simulink model "Stampfly_Tx"  (R2026b)
settings: Solver=FixedStepDiscrete  StopTime=inf  FixedStep=Official.Step
PostLoadFcn:
  | run(fullfile(fileparts(get_param('Stampfly_Tx','FileName')),'config','startup.m'));
InitFcn:
  | init_imu_flight;
undefined symbols (not defined in the file or in its folder): Official
libraries: slpidlib x7, simulink x4, mspfiltlib x1
(part 3 of 5)

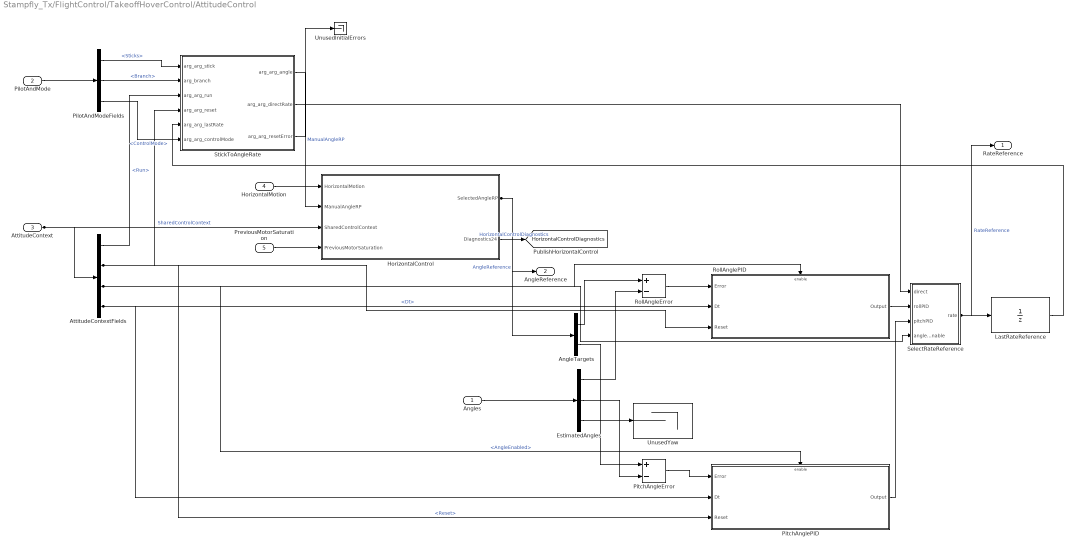
== system Stampfly_Tx/FlightControl/TakeoffHoverControl/AttitudeControl ==
  Angles : Inport
  PilotAndMode : Inport  Port=2
  AttitudeContext : Inport  Port=3
  HorizontalMotion : Inport  Description=HorizontalMotion：水平推定・制御のデータと実行条件を選択・結合します。2軸の順序は局所X（基準機首）、Y（右）です。  Port=4  OutDataTypeStr=Bus: HorizontalMotionBus
  PreviousMotorSaturation : Inport  Description=PreviousMotorSaturation：水平推定・制御のデータと実行条件を選択・結合します。2軸の順序は局所X（基準機首）、Y（右）です。  Port=5  OutDataTypeStr=boolean
  AngleTargets : Demux  Description=AngleTargets：ベクトルを元の成分順に分解します。個別の誤差や符号処理が必要な箇所で使います。  Outputs=2
  AttitudeContextFields : BusSelector  Description=AttitudeContextFields：バスから ControlContext.Run,ControlContext.Reset,ControlContext.AngleEnabled,Dt を選びます。元のベクトルの成分順序は変更しません。  OutputSignals=ControlContext.Run,ControlContext.Reset,ControlContext.AngleEnabled,Dt
  EstimatedAngles : Demux  Description=EstimatedAngles：ベクトルを元の成分順に分解します。個別の誤差や符号処理が必要な箇所で使います。  Outputs=3
  HorizontalControl : Subsystem  Description=HorizontalControl：水平推定・制御のデータと実行条件を選択・結合します。2軸の順序は局所X（基準機首）、Y（右）です。
      mask help: 水平制御：移動・減速・停止位置保持の速度目標、速度PI、姿勢目標への変換を行います。既存の姿勢・角速度PIDの前段です。
      mask Display: disp('HorizontalControl');port_label('input',1,'HorizontalMotion');port_label('input',2,'ManualAngleRP');port_label('input',3,'SharedControlContext');port_label('input',4,'PreviousMotorSaturation');port_label('output',1,'SelectedAngleRP');port_label('output',2,'Diagnostics24');
  LastRateReference : UnitDelay  Description=LastRateReference：前周期の値を保持して出力します。更新順序と状態保持に必要な 1 周期遅延です。初期値 zeros(3,1,'single')、周期 Official.Step 秒。  InitialCondition=zeros(3,1,'single')  SampleTime=Official.Step
  PilotAndModeFields : BusSelector  Description=PilotAndModeFields：バスから PilotInput.Sticks,SharedControlContext.FlightContext.Branch,SharedControlContext.ControlMode を選びます。元のベクトルの成分順序は変更しません。  OutputSignals=PilotInput.Sticks,SharedControlContext.FlightContext.Branch,SharedControlContext.ControlMode
  PitchAngleError : Sum  Description=PitchAngleError：入力を +- の符号で加減算します。ベクトルでは各成分に同じ演算を適用します。  Inputs=+-
  PitchAnglePID : Subsystem  Description=Pitch 角度 PID：角度誤差 [rad]→Pitch 角速度目標 [rad/s]。Stabilize 時の Enabled 境界と低推力 Reset を保ちます。
      mask help: Pitch 角度 PID：角度誤差 [rad]→Pitch 角速度目標 [rad/s]。Stabilize 時の Enabled 境界と低推力 Reset を保ちます。
      mask Display: disp('PitchAnglePID');port_label('input',1,'Error');port_label('input',2,'Dt');port_label('input',3,'Reset');port_label('output',1,'Output');
  RollAngleError : Sum  Description=RollAngleError：入力を +- の符号で加減算します。ベクトルでは各成分に同じ演算を適用します。  Inputs=+-
  RollAnglePID : Subsystem  Description=Roll 角度 PID：角度誤差 [rad]→Roll 角速度目標 [rad/s]。Stabilize 時の Enabled 境界と低推力 Reset を保ちます。
      mask help: Roll 角度 PID：角度誤差 [rad]→Roll 角速度目標 [rad/s]。Stabilize 時の Enabled 境界と低推力 Reset を保ちます。
      mask Display: disp('RollAnglePID');port_label('input',1,'Error');port_label('input',2,'Dt');port_label('input',3,'Reset');port_label('output',1,'Output');
  SelectRateReference : MATLAB Function  Description=角速度 PID の目標 [Roll, Pitch, Yaw] を選びます。Stabilize で角度制御が有効なときだけ Roll/Pitch を角度 PID の出力へ置換し、Yaw と Sport の直接角速度目標はそのまま使います。  TreatAsAtomicUnit=on
  StickToAngleRate : MATLAB Function  Description=操縦スティックから角度・角速度目標を作ります。Stabilize は Roll/Pitch ±30°、Sport は非線形な角速度指令、Yaw は角速度指令です。低推力リセット時に中立値を記憶します。  TreatAsAtomicUnit=on
  UnusedInitialErrors : Terminator
      settings: Description=操縦指令の既存関数が返す初期誤差を終端します。DedicatedPID の Reset により内部誤差を管理します。
  UnusedYaw : Terminator
      settings: Description=UnusedYaw：使用しない観測出力をここで終端します。接続された制御信号を変更しません。
  RateReference : Outport
  AngleReference : Outport  Port=2
  tag scope: HorizontalControlDiagnostics=global
  wires:
  Angles/1 -> EstimatedAngles/1
  AttitudeContextFields/2 -> PitchAnglePID/3(Reset), StickToAngleRate/4(arg_arg_reset), RollAnglePID/3(Reset)  "<Reset>"
  AttitudeContext/1 -> AttitudeContextFields/1, HorizontalControl/3(SharedControlContext)  "SharedControlContext"
  AttitudeContextFields/4 -> PitchAnglePID/2(Dt), RollAnglePID/2(Dt)  "<Dt>"
  PilotAndMode/1 -> PilotAndModeFields/1
  PilotAndModeFields/3 -> StickToAngleRate/6(arg_arg_controlMode)  "<ControlMode>"
  PilotAndModeFields/1 -> StickToAngleRate/1(arg_arg_stick)  "<Sticks>"
  PilotAndModeFields/2 -> StickToAngleRate/2(arg_branch)  "<Branch>"
  AttitudeContextFields/3 -> PitchAnglePID/Enable, SelectRateReference/4(angleEnable), RollAnglePID/Enable  "<AngleEnabled>"
  AttitudeContextFields/1 -> StickToAngleRate/3(arg_arg_run)  "<Run>"
  StickToAngleRate/1(arg_arg_angle) -> HorizontalControl/2(ManualAngleRP)  "ManualAngleRP"
  StickToAngleRate/2(arg_arg_directRate) -> SelectRateReference/1(direct)
  StickToAngleRate/3(arg_arg_resetError) -> UnusedInitialErrors/1
  EstimatedAngles/2 -> PitchAngleError/2
  HorizontalMotion/1 -> HorizontalControl/1(HorizontalMotion)
  RollAnglePID/1(Output) -> SelectRateReference/2(rollPID)
  PreviousMotorSaturation/1 -> HorizontalControl/4(PreviousMotorSaturation)
  HorizontalControl/1(SelectedAngleRP) -> AngleReference/1, AngleTargets/1  "AngleReference"
  HorizontalControl/2(Diagnostics24) -> [HorizontalControlDiagnostics]  "HorizontalControlDiagnostics"
  AngleTargets/1 -> RollAngleError/1
  AngleTargets/2 -> PitchAngleError/1
  SelectRateReference/1(rate) -> LastRateReference/1, RateReference/1  "RateReference"
  EstimatedAngles/1 -> RollAngleError/2
  EstimatedAngles/3 -> UnusedYaw/1
  RollAngleError/1 -> RollAnglePID/1(Error)
  PitchAngleError/1 -> PitchAnglePID/1(Error)
  PitchAnglePID/1(Output) -> SelectRateReference/3(pitchPID)
  LastRateReference/1 -> StickToAngleRate/5(arg_arg_lastRate)

== system Stampfly_Tx/FlightControl/TakeoffHoverControl/BodyRateControl ==
  RateReference : Inport
  MeasuredRates : Inport  Port=2
  RateContext : Inport  Port=3
  EstimatedRates : Demux  Description=EstimatedRates：ベクトルを元の成分順に分解します。個別の誤差や符号処理が必要な箇所で使います。  Outputs=3
  PitchRateError : Sum  Description=PitchRateError：入力を +- の符号で加減算します。ベクトルでは各成分に同じ演算を適用します。  Inputs=+-
  PitchRatePID : Subsystem  Description=Pitch 角速度 PID：角速度誤差 [rad/s]→Pitch のモーター補正。積分状態は Enable と Reset で管理し、実測 dt を入力します。
      mask help: Pitch 角速度 PID：角速度誤差 [rad/s]→Pitch のモーター補正。積分状態は Enable と Reset で管理し、実測 dt を入力します。
      mask Display: disp('PitchRatePID');port_label('input',1,'Error');port_label('input',2,'Dt');port_label('input',3,'Reset');port_label('output',1,'Output');
  RateContextFields : BusSelector  Description=制御の実行・リセット条件と実測 dt を選びます。DedicatedPID 内部で前回誤差を保持するため、未使用の PreviousError は取り出しません。  OutputSignals=ControlContext.Run,ControlContext.Reset,Dt
  RollRateError : Sum  Description=RollRateError：入力を +- の符号で加減算します。ベクトルでは各成分に同じ演算を適用します。  Inputs=+-
  RollRatePID : Subsystem  Description=Roll 角速度 PID：角速度誤差 [rad/s]→Roll のモーター補正。積分状態は Enable と Reset で管理し、実測 dt を入力します。
      mask help: Roll 角速度 PID：角速度誤差 [rad/s]→Roll のモーター補正。積分状態は Enable と Reset で管理し、実測 dt を入力します。
      mask Display: disp('RollRatePID');port_label('input',1,'Error');port_label('input',2,'Dt');port_label('input',3,'Reset');port_label('output',1,'Output');
  TargetRates : Demux  Description=TargetRates：ベクトルを元の成分順に分解します。個別の誤差や符号処理が必要な箇所で使います。  Outputs=3
  YawRateError : Sum  Description=YawRateError：入力を +- の符号で加減算します。ベクトルでは各成分に同じ演算を適用します。  Inputs=+-
  YawRatePID : Subsystem  Description=Yaw 角速度 PID：角速度誤差 [rad/s]→Yaw のモーター補正。Yaw の絶対角度制御は行わず、スティックの角速度目標を使います。
      mask help: Yaw 角速度 PID：角速度誤差 [rad/s]→Yaw のモーター補正。Yaw の絶対角度制御は行わず、スティックの角速度目標を使います。
      mask Display: disp('YawRatePID');port_label('input',1,'Error');port_label('input',2,'Dt');port_label('input',3,'Reset');port_label('output',1,'Output');
  RollTorque : Outport
  PitchTorque : Outport  Port=2
  YawTorque : Outport  Port=3
  wires:
  EstimatedRates/2 -> PitchRateError/2
  MeasuredRates/1 -> EstimatedRates/1
  RateReference/1 -> TargetRates/1
  TargetRates/3 -> YawRateError/1
  TargetRates/1 -> RollRateError/1
  TargetRates/2 -> PitchRateError/1
  EstimatedRates/3 -> YawRateError/2
  EstimatedRates/1 -> RollRateError/2
  RateContext/1 -> RateContextFields/1
  RollRateError/1 -> RollRatePID/1(Error)
  PitchRateError/1 -> PitchRatePID/1(Error)
  YawRateError/1 -> YawRatePID/1(Error)
  RateContextFields/1 -> YawRatePID/Enable, RollRatePID/Enable, PitchRatePID/Enable  "<Run>"
  RateContextFields/2 -> PitchRatePID/3(Reset), RollRatePID/3(Reset), YawRatePID/3(Reset)  "<Reset>"
  RateContextFields/3 -> YawRatePID/2(Dt), RollRatePID/2(Dt), PitchRatePID/2(Dt)  "<Dt>"
  RollRatePID/1(Output) -> RollTorque/1  "RollTorque"
  PitchRatePID/1(Output) -> PitchTorque/1  "PitchTorque"
  YawRatePID/1(Output) -> YawTorque/1  "YawTorque"

== system Stampfly_Tx/FlightControl/TakeoffHoverControl/FlightCommand ==
  PilotInput : Inport
  Height : Inport  Port=2
  FlightContext : Inport  Port=3
  TimingAndThrust : Inport  Port=4
  CommandStatusBus : BusCreator  Description=CommandStatusBus：異なる単位・型を持つ関連信号を名前付きバスにまとめます。入力線の信号名が項目名です。  Inputs=2
  ControlGating : Subsystem  Description=共通推力と飛行分岐から、全体・高度・角度・鉛直速度 PID の実行条件とリセットを決めます。制御の積分状態を校正・待機中に進めないための条件です。
      mask help: 共通推力と飛行分岐から、全体・高度・角度・鉛直速度 PID の実行条件とリセットを決めます。制御の積分状態を校正・待機中に進めないための条件です。
      mask Display: disp('ControlGating');port_label('input',1,'CommandMode');port_label('input',2,'ModeContext');port_label('input',3,'ThrustState');port_label('output',1,'ThrustRequest');port_label('output',2,'ControlContext');
  FinalizeFlightMode : Stateflow chart  Description=離着陸カウンターと制御状態から、周期末のモード・接続状態などを確定します。次周期に渡すモードと最上位の分岐を区別します。  TreatAsAtomicUnit=on
      mask help: 離着陸カウンターと制御状態から、周期末のモード・接続状態などを確定します。次周期に渡すモードと最上位の分岐を区別します。
  FlightCommandBus : BusCreator  Description=FlightCommandBus：異なる単位・型を持つ関連信号を名前付きバスにまとめます。入力線の信号名が項目名です。  Inputs=7
  FlightContextFields : BusSelector  Description=FlightContextFields：バスから Branch,PreMode を選びます。元のベクトルの成分順序は変更しません。  OutputSignals=Branch,PreMode
  ModeContextBus : BusCreator  Description=ModeContextBus：異なる単位・型を持つ関連信号を名前付きバスにまとめます。入力線の信号名が項目名です。  Inputs=3
  PilotInputFields : BusSelector  Description=PilotInputFields：バスから Sticks,BatteryVoltage,RangeFlag,OverG を選びます。元のベクトルの成分順序は変更しません。  OutputSignals=Sticks,BatteryVoltage,RangeFlag,OverG
  SharedControlContextBus : BusCreator  Description=SharedControlContextBus：異なる単位・型を持つ関連信号を名前付きバスにまとめます。入力線の信号名が項目名です。  Inputs=8
  TakeoffLandingCommand : Stateflow chart  Description=離陸・着陸、0.5 m の初期高度目標、0.05～1.8 m の高さ設定、基準推力と電圧トリムを状態として管理する Stateflow です。  TreatAsAtomicUnit=on
      mask help: 離陸・着陸、0.5 m の初期高度目標、0.05～1.8 m の高さ設定、基準推力と電圧トリムを状態として管理する Stateflow です。
  TimingAndThrustFields : BusSelector  Description=TimingAndThrustFields：バスから Dt,ThrustState を選びます。元のベクトルの成分順序は変更しません。  OutputSignals=Dt,ThrustState
  Zero : Constant  Description=Zero：固定値 single(0) を出力します。意味と単位は親の機能説明と信号名を参照します。  Value=single(0)
  FlightCommand : Outport
  SharedControlContext : Outport  Port=2
  CommandStatus : Outport  Port=3
  wires:
  ModeContextBus/1 -> ControlGating/2(ModeContext)  "ModeContext"
  Height/1 -> FinalizeFlightMode/3(height), TakeoffLandingCommand/2(height)
  TimingAndThrust/1 -> TimingAndThrustFields/1
  ControlGating/2(ControlContext) -> SharedControlContextBus/1  "ControlContext"
  PilotInput/1 -> SharedControlContextBus/3, PilotInputFields/1  "PilotInput"
  TakeoffLandingCommand/7(controlMode) -> SharedControlContextBus/8, FlightCommandBus/7  "ControlMode"
  FlightContext/1 -> ModeContextBus/1, SharedControlContextBus/2, FlightContextFields/1  "FlightContext"
  TakeoffLandingCommand/4(raw) -> FlightCommandBus/4  "RawThrust"
  FlightContextFields/1 -> TakeoffLandingCommand/5(mode), FinalizeFlightMode/1(branch)  "<Branch>"
  PilotInputFields/1 -> TakeoffLandingCommand/1(stick)  "<Sticks>"
  TakeoffLandingCommand/5(auto) -> FlightCommandBus/5, CommandStatusBus/1  "AltitudeEnabled"
  FlightContextFields/2 -> FinalizeFlightMode/2(preMode)  "<PreMode>"
  PilotInputFields/2 -> TakeoffLandingCommand/3(voltage)  "<BatteryVoltage>"
  PilotInputFields/3 -> TakeoffLandingCommand/4(rangeFlag)  "<RangeFlag>"
  PilotInputFields/4 -> FinalizeFlightMode/4(overG)  "<OverG>"
  TimingAndThrustFields/1 -> SharedControlContextBus/5, ModeContextBus/3  "<Dt>"
  TimingAndThrustFields/2 -> ControlGating/3(ThrustState)  "<ThrustState>"
  FinalizeFlightMode/1(mode) -> SharedControlContextBus/4, CommandStatusBus/2, ModeContextBus/2  "Mode"
  ControlGating/1(ThrustRequest) -> SharedControlContextBus/7  "ThrustRequest"
  TakeoffLandingCommand/1(alt) -> FlightCommandBus/1  "HeightReference"
  TakeoffLandingCommand/2(base) -> FlightCommandBus/2  "BaseThrust"
  TakeoffLandingCommand/3(counter) -> FlightCommandBus/3  "RampCounter"
  TakeoffLandingCommand/6(manual) -> FlightCommandBus/6  "ManualAltitude"
  FlightCommandBus/1 -> ControlGating/1(CommandMode), FlightCommand/1  "FlightCommand"
  CommandStatusBus/1 -> CommandStatus/1  "CommandStatus"
  Zero/1 -> SharedControlContextBus/6  "PreviousError"
  SharedControlContextBus/1 -> SharedControlContext/1  "SharedControlContext"

== system Stampfly_Tx/FlightControl/TakeoffHoverControl/FlightDiagnostics ==
  FlightCommand : Inport
  ControlReferences : Inport  Port=2
  MotorDiagnostics : Inport  Port=3
  ControlDiagnosticPack : MATLAB Function  Description=制御内部の観測値を 17 要素の single ベクトルにまとめます。ログの項目順は [高度制御状態; 基準推力; 離陸カウンター; 高度目標; 推力; 角度目標2; 角速度目標3; 軸補正3; 配分前モーター値4] です。制御判断は行いません。  TreatAsAtomicUnit=on
  ControlReferencesFields : BusSelector  Description=ControlReferencesFields：バスから VelocityReference,Thrust,Angles,RateReference を選びます。元のベクトルの成分順序は変更しません。  OutputSignals=VelocityReference,Thrust,Angles,RateReference
  FlightCommandFields : BusSelector  Description=FlightCommandFields：バスから HeightReference,BaseThrust,RampCounter を選びます。元のベクトルの成分順序は変更しません。  OutputSignals=HeightReference,BaseThrust,RampCounter
  MotorDiagnosticsFields : BusSelector  Description=MotorDiagnosticsFields：バスから RollTorque,PitchTorque,YawTorque,BeforeLimit を選びます。元のベクトルの成分順序は変更しません。  OutputSignals=RollTorque,PitchTorque,YawTorque,BeforeLimit
  Diagnostics : Outport
  wires:
  MotorDiagnostics/1 -> MotorDiagnosticsFields/1
  FlightCommand/1 -> FlightCommandFields/1
  ControlReferences/1 -> ControlReferencesFields/1
  FlightCommandFields/1 -> ControlDiagnosticPack/1(alt)  "<HeightReference>"
  FlightCommandFields/2 -> ControlDiagnosticPack/2(base)  "<BaseThrust>"
  ControlReferencesFields/1 -> ControlDiagnosticPack/4(zRef)  "<VelocityReference>"
  FlightCommandFields/3 -> ControlDiagnosticPack/3(counter)  "<RampCounter>"
  ControlReferencesFields/2 -> ControlDiagnosticPack/5(thrust)  "<Thrust>"
  ControlReferencesFields/3 -> ControlDiagnosticPack/6(angle)  "<Angles>"
  ControlReferencesFields/4 -> ControlDiagnosticPack/7(rate)  "<RateReference>"
  MotorDiagnosticsFields/1 -> ControlDiagnosticPack/8(rollTorque)  "<RollTorque>"
  MotorDiagnosticsFields/2 -> ControlDiagnosticPack/9(pitchTorque)  "<PitchTorque>"
  MotorDiagnosticsFields/3 -> ControlDiagnosticPack/10(yawTorque)  "<YawTorque>"
  MotorDiagnosticsFields/4 -> ControlDiagnosticPack/11(before)  "<BeforeLimit>"
  ControlDiagnosticPack/1(diag) -> Diagnostics/1  "Diagnostics"

== system Stampfly_Tx/FlightControl/TakeoffHoverControl/JapaneseExplanation ==

== system Stampfly_Tx/FlightControl/TakeoffHoverControl/MotorAllocation ==
  MotorEffort : Inport
  MotorContext : Inport  Port=2
  MotorCommandBus : BusCreator  Description=MotorCommandBus：異なる単位・型を持つ関連信号を名前付きバスにまとめます。入力線の信号名が項目名です。  Inputs=2
  MotorContextFields : BusSelector  Description=MotorContextFields：バスから ControlContext.Run,ControlContext.Reset,PilotInput.OverG,FlightContext.Branch,Dt を選びます。元のベクトルの成分順序は変更しません。  OutputSignals=ControlContext.Run,ControlContext.Reset,PilotInput.OverG,FlightContext.Branch,Dt
  MotorEffortFields : BusSelector  Description=MotorEffortFields：バスから Thrust,RollTorque,PitchTorque,YawTorque を選びます。元のベクトルの成分順序は変更しません。  OutputSignals=Thrust,RollTorque,PitchTorque,YawTorque
  MotorMixerFilter8bit : Subsystem  Description=4 モーターの符号付き配分、平滑化、飽和、8 bit 変換を一連の処理として示します。モーター順 [FR, FL, RR, RL] は出力・ログでも同じです。
      mask help: 4 モーターの符号付き配分、平滑化、飽和、8 bit 変換を一連の処理として示します。モーター順 [FR, FL, RR, RL] は出力・ログでも同じです。
      mask Display: disp('MotorMixerFilter8bit');port_label('input',1,'Thrust');port_label('input',2,'RollTorque');port_label('input',3,'PitchTorque');port_label('input',4,'YawTorque');port_label('input',5,'Run');port_label('input',6,'Reset');port_label('input',7,'OverG');port_label('input',8,'Mode');port_label('input',9,'Dt');port_label('output',1,'Duty4');port_label('output',2,'Counts4');port_label('output',3,'BeforeLimit4');
  MotorCommand : Outport
  BeforeLimit : Outport  Port=2
  wires:
  MotorEffortFields/1 -> MotorMixerFilter8bit/1(Thrust)  "<Thrust>"
  MotorMixerFilter8bit/3(BeforeLimit4) -> BeforeLimit/1  "BeforeLimit"
  MotorEffort/1 -> MotorEffortFields/1
  MotorContextFields/2 -> MotorMixerFilter8bit/6(Reset)  "<Reset>"
  MotorEffortFields/3 -> MotorMixerFilter8bit/3(PitchTorque)  "<PitchTorque>"
  MotorContext/1 -> MotorContextFields/1
  MotorContextFields/1 -> MotorMixerFilter8bit/5(Run)  "<Run>"
  MotorEffortFields/2 -> MotorMixerFilter8bit/2(RollTorque)  "<RollTorque>"
  MotorEffortFields/4 -> MotorMixerFilter8bit/4(YawTorque)  "<YawTorque>"
  MotorContextFields/3 -> MotorMixerFilter8bit/7(OverG)  "<OverG>"
  MotorContextFields/4 -> MotorMixerFilter8bit/8(Mode)  "<Branch>"
  MotorContextFields/5 -> MotorMixerFilter8bit/9(Dt)  "<Dt>"
  MotorMixerFilter8bit/1(Duty4) -> MotorCommandBus/1  "Duty"
  MotorMixerFilter8bit/2(Counts4) -> MotorCommandBus/2  "Counts"
  MotorCommandBus/1 -> MotorCommand/1  "MotorCommand"

== system Stampfly_Tx/SensorCorrection/IMUAxisConversion/JapaneseExplanation ==

== system Stampfly_Tx/SensorCorrection/IMUFiltering/AccelLowpassXYZ ==
  Input : Inport  PortDimensions=3
  Dt : Inport  Port=2
  Reset : Inport  Port=3
  Enable : Inport  Port=4
  Denominator : Sum  Description=Denominator：入力を ++ の符号で加減算します。ベクトルでは各成分に同じ演算を適用します。
  InputTerm : Product  Description=InputTerm：入力の乗算・除算（*/）を行います。フィルターは既存の演算順序を保ちます。  Inputs=*/
  InputTimesDt : Product  Description=InputTimesDt：入力の乗算・除算（**）を行います。フィルターは既存の演算順序を保ちます。  Inputs=**
  PreviousFiltered : UnitDelay  Description=PreviousFiltered：前周期の値を保持して出力します。更新順序と状態保持に必要な 1 周期遅延です。初期値 zeros(3,1,'single')、周期 .0025 秒。  InitialCondition=zeros(3,1,'single')  SampleTime=.0025
  PreviousTerm : Product  Description=PreviousTerm：入力の乗算・除算（*/）を行います。フィルターは既存の演算順序を保ちます。  Inputs=*/
  PreviousTimesT : Product  Description=PreviousTimesT：入力の乗算・除算（**）を行います。フィルターは既存の演算順序を保ちます。  Inputs=**
  ResetPrevious : Switch  Description=ResetPrevious：条件入力で更新値と保持・リセット値を選びます。条件は u2 ~= 0。  Criteria=u2 ~= 0  SaturateOnIntegerOverflow=off  InputSameDT=off
  TimeConstantS : Constant  Description=TimeConstantS：固定値 single(0.0030000000000000001) を出力します。意味と単位は親の機能説明と信号名を参照します。  Value=single(0.0030000000000000001)
  UpdateOrHold : Switch  Description=UpdateOrHold：条件入力で更新値と保持・リセット値を選びます。条件は u2 ~= 0。  Criteria=u2 ~= 0  SaturateOnIntegerOverflow=off  InputSameDT=off
  UpdatedFiltered : Sum  Description=UpdatedFiltered：入力を ++ の符号で加減算します。ベクトルでは各成分に同じ演算を適用します。
  ZeroOnReset : Constant  Description=ZeroOnReset：固定値 zeros(3,1,'single') を出力します。意味と単位は親の機能説明と信号名を参照します。  Value=zeros(3,1,'single')
  Filtered : Outport
  wires:
  Reset/1 -> ResetPrevious/2
  TimeConstantS/1 -> PreviousTimesT/2, Denominator/1
  Input/1 -> InputTimesDt/1
  Enable/1 -> UpdateOrHold/2
  InputTerm/1 -> UpdatedFiltered/2
  Denominator/1 -> PreviousTerm/2, InputTerm/2
  InputTimesDt/1 -> InputTerm/1
  ResetPrevious/1 -> UpdateOrHold/3, PreviousTimesT/1
  Dt/1 -> Denominator/2, InputTimesDt/2
  UpdatedFiltered/1 -> UpdateOrHold/1
  UpdateOrHold/1 -> PreviousFiltered/1, Filtered/1
  ZeroOnReset/1 -> ResetPrevious/1
  PreviousFiltered/1 -> ResetPrevious/3
  PreviousTimesT/1 -> PreviousTerm/1
  PreviousTerm/1 -> UpdatedFiltered/1

== system Stampfly_Tx/SensorCorrection/IMUFiltering/GyroLowpassXYZ ==
  Input : Inport  PortDimensions=3
  Dt : Inport  Port=2
  Reset : Inport  Port=3
  Enable : Inport  Port=4
  Denominator : Sum  Description=Denominator：入力を ++ の符号で加減算します。ベクトルでは各成分に同じ演算を適用します。
  InputTerm : Product  Description=InputTerm：入力の乗算・除算（*/）を行います。フィルターは既存の演算順序を保ちます。  Inputs=*/
  InputTimesDt : Product  Description=InputTimesDt：入力の乗算・除算（**）を行います。フィルターは既存の演算順序を保ちます。  Inputs=**
  PreviousFiltered : UnitDelay  Description=PreviousFiltered：前周期の値を保持して出力します。更新順序と状態保持に必要な 1 周期遅延です。初期値 zeros(3,1,'single')、周期 .0025 秒。  InitialCondition=zeros(3,1,'single')  SampleTime=.0025
  PreviousTerm : Product  Description=PreviousTerm：入力の乗算・除算（*/）を行います。フィルターは既存の演算順序を保ちます。  Inputs=*/
  PreviousTimesT : Product  Description=PreviousTimesT：入力の乗算・除算（**）を行います。フィルターは既存の演算順序を保ちます。  Inputs=**
  ResetPrevious : Switch  Description=ResetPrevious：条件入力で更新値と保持・リセット値を選びます。条件は u2 ~= 0。  Criteria=u2 ~= 0  SaturateOnIntegerOverflow=off  InputSameDT=off
  TimeConstantS : Constant  Description=TimeConstantS：固定値 single(0.0030000000000000001) を出力します。意味と単位は親の機能説明と信号名を参照します。  Value=single(0.0030000000000000001)
  UpdateOrHold : Switch  Description=UpdateOrHold：条件入力で更新値と保持・リセット値を選びます。条件は u2 ~= 0。  Criteria=u2 ~= 0  SaturateOnIntegerOverflow=off  InputSameDT=off
  UpdatedFiltered : Sum  Description=UpdatedFiltered：入力を ++ の符号で加減算します。ベクトルでは各成分に同じ演算を適用します。
  ZeroOnReset : Constant  Description=ZeroOnReset：固定値 zeros(3,1,'single') を出力します。意味と単位は親の機能説明と信号名を参照します。  Value=zeros(3,1,'single')
  Filtered : Outport
  wires:
  Reset/1 -> ResetPrevious/2
  TimeConstantS/1 -> PreviousTimesT/2, Denominator/1
  Input/1 -> InputTimesDt/1
  Enable/1 -> UpdateOrHold/2
  InputTerm/1 -> UpdatedFiltered/2
  Denominator/1 -> PreviousTerm/2, InputTerm/2
  InputTimesDt/1 -> InputTerm/1
  ResetPrevious/1 -> UpdateOrHold/3, PreviousTimesT/1
  Dt/1 -> InputTimesDt/2, Denominator/2
  UpdatedFiltered/1 -> UpdateOrHold/1
  UpdateOrHold/1 -> Filtered/1, PreviousFiltered/1
  ZeroOnReset/1 -> ResetPrevious/1
  PreviousFiltered/1 -> ResetPrevious/3
  PreviousTimesT/1 -> PreviousTerm/1
  PreviousTerm/1 -> UpdatedFiltered/1

== system Stampfly_Tx/SensorCorrection/IMUFiltering/JapaneseExplanation ==

== system Stampfly_Tx/SensorCorrection/IMUFiltering/VerticalDeltaLowpass ==
  Input : Inport
  Dt : Inport  Port=2
  Reset : Inport  Port=3
  Enable : Inport  Port=4
  Denominator : Sum  Description=Denominator：入力を ++ の符号で加減算します。ベクトルでは各成分に同じ演算を適用します。
  InputTerm : Product  Description=InputTerm：入力の乗算・除算（*/）を行います。フィルターは既存の演算順序を保ちます。  Inputs=*/
  InputTimesDt : Product  Description=InputTimesDt：入力の乗算・除算（**）を行います。フィルターは既存の演算順序を保ちます。  Inputs=**
  PreviousFiltered : UnitDelay  Description=PreviousFiltered：前周期の値を保持して出力します。更新順序と状態保持に必要な 1 周期遅延です。初期値 single(0)、周期 .0025 秒。  InitialCondition=single(0)  SampleTime=.0025
  PreviousTerm : Product  Description=PreviousTerm：入力の乗算・除算（*/）を行います。フィルターは既存の演算順序を保ちます。  Inputs=*/
  PreviousTimesT : Product  Description=PreviousTimesT：入力の乗算・除算（**）を行います。フィルターは既存の演算順序を保ちます。  Inputs=**
  ResetPrevious : Switch  Description=ResetPrevious：条件入力で更新値と保持・リセット値を選びます。条件は u2 ~= 0。  Criteria=u2 ~= 0  SaturateOnIntegerOverflow=off  InputSameDT=off
  TimeConstantS : Constant  Description=TimeConstantS：固定値 single(0.10000000000000001) を出力します。意味と単位は親の機能説明と信号名を参照します。  Value=single(0.10000000000000001)
  UpdateOrHold : Switch  Description=UpdateOrHold：条件入力で更新値と保持・リセット値を選びます。条件は u2 ~= 0。  Criteria=u2 ~= 0  SaturateOnIntegerOverflow=off  InputSameDT=off
  UpdatedFiltered : Sum  Description=UpdatedFiltered：入力を ++ の符号で加減算します。ベクトルでは各成分に同じ演算を適用します。
  ZeroOnReset : Constant  Description=ZeroOnReset：固定値 single(0) を出力します。意味と単位は親の機能説明と信号名を参照します。  Value=single(0)
  Filtered : Outport
  wires:
  Reset/1 -> ResetPrevious/2
  TimeConstantS/1 -> PreviousTimesT/2, Denominator/1
  Input/1 -> InputTimesDt/1
  Enable/1 -> UpdateOrHold/2
  InputTerm/1 -> UpdatedFiltered/2
  Denominator/1 -> PreviousTerm/2, InputTerm/2
  InputTimesDt/1 -> InputTerm/1
  ResetPrevious/1 -> UpdateOrHold/3, PreviousTimesT/1
  Dt/1 -> Denominator/2, InputTimesDt/2
  UpdatedFiltered/1 -> UpdateOrHold/1
  UpdateOrHold/1 -> PreviousFiltered/1, Filtered/1
  ZeroOnReset/1 -> ResetPrevious/1
  PreviousFiltered/1 -> ResetPrevious/3
  PreviousTimesT/1 -> PreviousTerm/1
  PreviousTerm/1 -> UpdatedFiltered/1

== system Stampfly_Tx/SensorCorrection/VerticalAcceleration/JapaneseExplanation ==

== system Stampfly_Tx/SensorCorrection/VerticalAcceleration/VerticalLowpass ==
  Input : Inport
  Dt : Inport  Port=2
  Reset : Inport  Port=3
  Enable : Inport  Port=4
  Denominator : Sum  Description=Denominator：入力を ++ の符号で加減算します。ベクトルでは各成分に同じ演算を適用します。
  InputTerm : Product  Description=InputTerm：入力の乗算・除算（*/）を行います。フィルターは既存の演算順序を保ちます。  Inputs=*/
  InputTimesDt : Product  Description=InputTimesDt：入力の乗算・除算（**）を行います。フィルターは既存の演算順序を保ちます。  Inputs=**
  PreviousFiltered : UnitDelay  Description=PreviousFiltered：前周期の値を保持して出力します。更新順序と状態保持に必要な 1 周期遅延です。初期値 single(0)、周期 .0025 秒。  InitialCondition=single(0)  SampleTime=.0025
  PreviousTerm : Product  Description=PreviousTerm：入力の乗算・除算（*/）を行います。フィルターは既存の演算順序を保ちます。  Inputs=*/
  PreviousTimesT : Product  Description=PreviousTimesT：入力の乗算・除算（**）を行います。フィルターは既存の演算順序を保ちます。  Inputs=**
  ResetPrevious : Switch  Description=ResetPrevious：条件入力で更新値と保持・リセット値を選びます。条件は u2 ~= 0。  Criteria=u2 ~= 0  SaturateOnIntegerOverflow=off  InputSameDT=off
  TimeConstantS : Constant  Description=TimeConstantS：固定値 single(0.10000000000000001) を出力します。意味と単位は親の機能説明と信号名を参照します。  Value=single(0.10000000000000001)
  UpdateOrHold : Switch  Description=UpdateOrHold：条件入力で更新値と保持・リセット値を選びます。条件は u2 ~= 0。  Criteria=u2 ~= 0  SaturateOnIntegerOverflow=off  InputSameDT=off
  UpdatedFiltered : Sum  Description=UpdatedFiltered：入力を ++ の符号で加減算します。ベクトルでは各成分に同じ演算を適用します。
  ZeroOnReset : Constant  Description=ZeroOnReset：固定値 single(0) を出力します。意味と単位は親の機能説明と信号名を参照します。  Value=single(0)
  Filtered : Outport
  wires:
  Reset/1 -> ResetPrevious/2
  TimeConstantS/1 -> Denominator/1, PreviousTimesT/2
  Input/1 -> InputTimesDt/1
  Enable/1 -> UpdateOrHold/2
  InputTerm/1 -> UpdatedFiltered/2
  Denominator/1 -> PreviousTerm/2, InputTerm/2
  InputTimesDt/1 -> InputTerm/1
  ResetPrevious/1 -> UpdateOrHold/3, PreviousTimesT/1
  Dt/1 -> InputTimesDt/2, Denominator/2
  UpdatedFiltered/1 -> UpdateOrHold/1
  UpdateOrHold/1 -> PreviousFiltered/1, Filtered/1
  ZeroOnReset/1 -> ResetPrevious/1
  PreviousFiltered/1 -> ResetPrevious/3
  PreviousTimesT/1 -> PreviousTerm/1
  PreviousTerm/1 -> UpdatedFiltered/1

== system Stampfly_Tx/AttitudeAltitudeEstimation/IMUAttitude/FusionState/UpdateWhenReady ==
  Accel : Inport  PortDimensions=[1 3]
  Gyro : Inport  Port=2  PortDimensions=[1 3]
  Reset : ResetPort  DisableCoverage=on  ResetTriggerType=level
  IMU Filter : mspfiltlib/IMU Filter  DispRefFrame=NED  OrientationFormat=quaternion  DecimationFactor=1  InitialProcessNoise=IMUFlight.InitialProcessNoise  AccelerometerNoise=IMUFlight.AccelerometerNoise  GyroscopeNoise=IMUFlight.GyroscopeNoise  GyroscopeDriftNoise=IMUFlight.GyroscopeDriftNoise  LinearAccelerationNoise=IMUFlight.LinearAccelerationNoise  LinearAccelerationDecayFactor=IMUFlight.LinearAccelerationDecayFactor  SimulateUsing=Code generation
  Orientation : Outport  PortDimensions=[1 4]  InitialOutput=single([1 0 0 0])
  AngularVelocity : Outport  Port=2  PortDimensions=[1 3]  InitialOutput=single([0 0 0])
  wires:
  IMU Filter/2 -> AngularVelocity/1
  IMU Filter/1 -> Orientation/1
  Gyro/1 -> IMU Filter/2
  Accel/1 -> IMU Filter/1

== system Stampfly_Tx/FlightControl/TakeoffHoverControl/AltitudeControl/AltitudePID ==
  Error : Inport
  Dt : Inport  Port=2
  Reset : Inport  Port=3
  Enable : EnablePort
  DedicatedPID : slpidlib/PID Controller  Description=飛行比較用の専用PID。Ideal形式、台形積分・微分フィルター、実測Dt、単精度。  Controller=PID  Form=Ideal  TimeDomain=Discrete-time  UseExternalTs=on  SampleTime=.0025  IntegratorMethod=Trapezoidal  FilterMethod=Trapezoidal  ControllerParametersSource=internal  P=single(0.37999999523162842)  I=single(1)/single(10)  UseKiTs=off  D=single(0.5)  UseExternalDerivativeSource=off  N=single(1)/(single(0.125)*single(0.5))  UseFilter=on  TunerSelectOption=Transfer Function Based (PID Tuner App)  InitialConditionSource=external  InitialConditionForIntegrator=0  InitialConditionForFilter=0  DifferentiatorICPrevScaledInput=0  ExternalReset=level  TrackingMode=off  Kt=1  LimitOutput=off  SatLimitsSource=internal  UpperSaturationLimit=inf  LowerSaturationLimit=-inf  LinearizeAsGain=off  AntiWindupMode=none  Kb=1  LimitIntegrator=on  UpperIntegratorSaturationLimit=single(30000)  LowerIntegratorSaturationLimit=single(-30000)  PGainOutDataTypeStr=single  PProdOutDataTypeStr=single  POutMin=[]  POutMax=[]  IGainOutDataTypeStr=single  IProdOutDataTypeStr=single  IOutMin=[]  IOutMax=[]  DGainOutDataTypeStr=single  DProdOutDataTypeStr=single  DOutMin=[]  DOutMax=[]  NGainOutDataTypeStr=single  NProdOutDataTypeStr=single  NOutMin=[]  NOutMax=[]  SumOutDataTypeStr=single  SumOutMin=[]  SumOutMax=[]  SaturationOutDataTypeStr=single  SaturationOutMin=[]  SaturationOutMax=[]  PParamDataTypeStr=single  PParamMin=[]  PParamMax=[]  IParamDataTypeStr=single  IParamMin=[]  IParamMax=[]  DParamDataTypeStr=single  DParamMin=[]  DParamMax=[]  NParamDataTypeStr=single  NParamMin=[]  NParamMax=[]  KbParamDataTypeStr=single  KbParamMin=[]  KbParamMax=[]  KtParamDataTypeStr=single  KtParamMin=[]  KtParamMax=[]  KbOutDataTypeStr=single  KbOutMin=[]  KbOutMax=[]  KtOutDataTypeStr=single  KtOutMin=[]  KtOutMax=[]  IntegratorOutDataTypeStr=single  IntegratorOutMin=[]  IntegratorOutMax=[]  FilterOutDataTypeStr=single  FilterOutMin=[]  FilterOutMax=[]  SumI1OutDataTypeStr=single  SumI1OutMin=[]  SumI1OutMax=[]  SumI2OutDataTypeStr=single  SumI2OutMin=[]  SumI2OutMax=[]  SumI3OutDataTypeStr=single  SumI3OutMin=[]  SumI3OutMax=[]  SumI4OutDataTypeStr=single  SumI4OutMin=[]  SumI4OutMax=[]  SumDOutDataTypeStr=single  SumDOutMin=[]  SumDOutMax=[]  SumAccumDataTypeStr=single  SumI1AccumDataTypeStr=single  SumI2AccumDataTypeStr=single  SumI3AccumDataTypeStr=single  SumI4AccumDataTypeStr=single  SumDAccumDataTypeStr=single  DifferentiatorOutDataTypeStr=single  DifferentiatorOutMin=[]  DifferentiatorOutMax=[]  FilterDiffOutCoefMin=[]  FilterDiffOutCoefMax=[]  ReciprocalOutDataTypeStr=single  ReciprocalOutMin=[]  ReciprocalOutMax=[]  SumDenOutDataTypeStr=single  SumDenOutMin=[]  SumDenOutMax=[]  SumNumOutDataTypeStr=single  SumNumOutMin=[]  SumNumOutMax=[]  SumDenAccumDataTypeStr=single  SumNumAccumDataTypeStr=single  DivideOutDataTypeStr=single  DivideOutMin=[]  DivideOutMax=[]  UdiffTsProdOutDataTypeStr=single  UdiffTsProdOutMin=[]  UdiffTsProdOutMax=[]  NTsProdOutDataTypeStr=single  NTsProdOutMin=[]  NTsProdOutMax=[]  UintegralTsProdOutDataTypeStr=single  UintegralTsProdOutMin=[]  UintegralTsProdOutMax=[]  UngainTsProdOutDataTypeStr=single  UngainTsProdOutMin=[]  UngainTsProdOutMax=[]  ClampingZeroOutDataTypeStr=single  ClampingZeroOutMin=[]  ClampingZeroOutMax=[]  FilterDenConstantOutDataTypeStr=single  FilterDenConstantOutMin=[]  FilterDenConstantOutMax=[]  PCopyOutDataTypeStr=single  PCopyOutMin=[]  PCopyOutMax=[]  NCopyOutDataTypeStr=single  NCopyOutMin=[]  NCopyOutMax=[]  IntegratorContinuousStateAttributes=''  IntegratorStateMustResolveToSignalObject=off  IntegratorRTWStateStorageClass=Auto  FilterContinuousStateAttributes=''  FilterStateMustResolveToSignalObject=off  FilterRTWStateStorageClass=Auto  ParallelPVariant=Passthrough  IdealPVariant=InternalParameters  IVariant=InternalParameters  DVariant=InternalParameters  IntegratorVariant=Discrete  SatVariant=Disabled  AWVariant=Passthrough  PCopyVariant=Disabled  TRVariant=Disabled  FdbkBlocksVariant=Forward  IdealPFdbkVariant=Disabled  SatFdbkVariant=Disabled  DerivativeFilterVariant=TrapezoidalFilter  NVariant=InternalParameters  NCopyVariant=InternalParameters  FilterICVariant=ExternalICs  IntegratorICVariant=ExternalICs  ExternalResetVariant=ExternalReset  TRSumVariant=Passthrough  SumFdbkVariant=Disabled  SumVariant=Sum_PID  TsampFilterVariant=ExternalTs  TsampNgainVariant=Passthrough  TsampIntegralVariant=ExternalTs  ExternalSaturationOutDataTypeStr=Inherit: Same as second input  DerivativeSourceVariant=ErrorSignal  PreIntVariant=InternalPreInt
      settings: LibrarySourceBlock=simulink/Discrete/Discrete PID Controller
  ZeroInitialCondition : Constant  Description=ZeroInitialCondition：固定値 single(0) を出力します。意味と単位は親の機能説明と信号名を参照します。  Value=single(0)
  Output : Outport
  wires:
  DedicatedPID/1 -> Output/1
  Dt/1 -> DedicatedPID/5
  ZeroInitialCondition/1 -> DedicatedPID/3, DedicatedPID/4
  Reset/1 -> DedicatedPID/2
  Error/1 -> DedicatedPID/1

== system Stampfly_Tx/FlightControl/TakeoffHoverControl/AltitudeControl/VerticalSpeedPID ==
  Error : Inport
  Dt : Inport  Port=2
  Reset : Inport  Port=3
  Enable : EnablePort
  DedicatedPID : slpidlib/PID Controller  Description=飛行比較用の専用PID。Ideal形式、台形積分・微分フィルター、実測Dt、単精度。  Controller=PID  Form=Ideal  TimeDomain=Discrete-time  UseExternalTs=on  SampleTime=.0025  IntegratorMethod=Trapezoidal  FilterMethod=Trapezoidal  ControllerParametersSource=internal  P=single(0.079999998211860657)  I=single(1)/single(0.94999998807907104)  UseKiTs=off  D=single(0.079999998211860657)  UseExternalDerivativeSource=off  N=single(1)/(single(0.125)*single(0.079999998211860657))  UseFilter=on  TunerSelectOption=Transfer Function Based (PID Tuner App)  InitialConditionSource=external  InitialConditionForIntegrator=0  InitialConditionForFilter=0  DifferentiatorICPrevScaledInput=0  ExternalReset=level  TrackingMode=off  Kt=1  LimitOutput=off  SatLimitsSource=internal  UpperSaturationLimit=inf  LowerSaturationLimit=-inf  LinearizeAsGain=off  AntiWindupMode=none  Kb=1  LimitIntegrator=on  UpperIntegratorSaturationLimit=single(30000)  LowerIntegratorSaturationLimit=single(-30000)  PGainOutDataTypeStr=single  PProdOutDataTypeStr=single  POutMin=[]  POutMax=[]  IGainOutDataTypeStr=single  IProdOutDataTypeStr=single  IOutMin=[]  IOutMax=[]  DGainOutDataTypeStr=single  DProdOutDataTypeStr=single  DOutMin=[]  DOutMax=[]  NGainOutDataTypeStr=single  NProdOutDataTypeStr=single  NOutMin=[]  NOutMax=[]  SumOutDataTypeStr=single  SumOutMin=[]  SumOutMax=[]  SaturationOutDataTypeStr=single  SaturationOutMin=[]  SaturationOutMax=[]  PParamDataTypeStr=single  PParamMin=[]  PParamMax=[]  IParamDataTypeStr=single  IParamMin=[]  IParamMax=[]  DParamDataTypeStr=single  DParamMin=[]  DParamMax=[]  NParamDataTypeStr=single  NParamMin=[]  NParamMax=[]  KbParamDataTypeStr=single  KbParamMin=[]  KbParamMax=[]  KtParamDataTypeStr=single  KtParamMin=[]  KtParamMax=[]  KbOutDataTypeStr=single  KbOutMin=[]  KbOutMax=[]  KtOutDataTypeStr=single  KtOutMin=[]  KtOutMax=[]  IntegratorOutDataTypeStr=single  IntegratorOutMin=[]  IntegratorOutMax=[]  FilterOutDataTypeStr=single  FilterOutMin=[]  FilterOutMax=[]  SumI1OutDataTypeStr=single  SumI1OutMin=[]  SumI1OutMax=[]  SumI2OutDataTypeStr=single  SumI2OutMin=[]  SumI2OutMax=[]  SumI3OutDataTypeStr=single  SumI3OutMin=[]  SumI3OutMax=[]  SumI4OutDataTypeStr=single  SumI4OutMin=[]  SumI4OutMax=[]  SumDOutDataTypeStr=single  SumDOutMin=[]  SumDOutMax=[]  SumAccumDataTypeStr=single  SumI1AccumDataTypeStr=single  SumI2AccumDataTypeStr=single  SumI3AccumDataTypeStr=single  SumI4AccumDataTypeStr=single  SumDAccumDataTypeStr=single  DifferentiatorOutDataTypeStr=single  DifferentiatorOutMin=[]  DifferentiatorOutMax=[]  FilterDiffOutCoefMin=[]  FilterDiffOutCoefMax=[]  ReciprocalOutDataTypeStr=single  ReciprocalOutMin=[]  ReciprocalOutMax=[]  SumDenOutDataTypeStr=single  SumDenOutMin=[]  SumDenOutMax=[]  SumNumOutDataTypeStr=single  SumNumOutMin=[]  SumNumOutMax=[]  SumDenAccumDataTypeStr=single  SumNumAccumDataTypeStr=single  DivideOutDataTypeStr=single  DivideOutMin=[]  DivideOutMax=[]  UdiffTsProdOutDataTypeStr=single  UdiffTsProdOutMin=[]  UdiffTsProdOutMax=[]  NTsProdOutDataTypeStr=single  NTsProdOutMin=[]  NTsProdOutMax=[]  UintegralTsProdOutDataTypeStr=single  UintegralTsProdOutMin=[]  UintegralTsProdOutMax=[]  UngainTsProdOutDataTypeStr=single  UngainTsProdOutMin=[]  UngainTsProdOutMax=[]  ClampingZeroOutDataTypeStr=single  ClampingZeroOutMin=[]  ClampingZeroOutMax=[]  FilterDenConstantOutDataTypeStr=single  FilterDenConstantOutMin=[]  FilterDenConstantOutMax=[]  PCopyOutDataTypeStr=single  PCopyOutMin=[]  PCopyOutMax=[]  NCopyOutDataTypeStr=single  NCopyOutMin=[]  NCopyOutMax=[]  IntegratorContinuousStateAttributes=''  IntegratorStateMustResolveToSignalObject=off  IntegratorRTWStateStorageClass=Auto  FilterContinuousStateAttributes=''  FilterStateMustResolveToSignalObject=off  FilterRTWStateStorageClass=Auto  ParallelPVariant=Passthrough  IdealPVariant=InternalParameters  IVariant=InternalParameters  DVariant=InternalParameters  IntegratorVariant=Discrete  SatVariant=Disabled  AWVariant=Passthrough  PCopyVariant=Disabled  TRVariant=Disabled  FdbkBlocksVariant=Forward  IdealPFdbkVariant=Disabled  SatFdbkVariant=Disabled  DerivativeFilterVariant=TrapezoidalFilter  NVariant=InternalParameters  NCopyVariant=InternalParameters  FilterICVariant=ExternalICs  IntegratorICVariant=ExternalICs  ExternalResetVariant=ExternalReset  TRSumVariant=Passthrough  SumFdbkVariant=Disabled  SumVariant=Sum_PID  TsampFilterVariant=ExternalTs  TsampNgainVariant=Passthrough  TsampIntegralVariant=ExternalTs  ExternalSaturationOutDataTypeStr=Inherit: Same as second input  DerivativeSourceVariant=ErrorSignal  PreIntVariant=InternalPreInt
      settings: LibrarySourceBlock=simulink/Discrete/Discrete PID Controller
  ZeroInitialCondition : Constant  Description=ZeroInitialCondition：固定値 single(0) を出力します。意味と単位は親の機能説明と信号名を参照します。  Value=single(0)
  Output : Outport
  wires:
  DedicatedPID/1 -> Output/1
  Dt/1 -> DedicatedPID/5
  ZeroInitialCondition/1 -> DedicatedPID/4, DedicatedPID/3
  Reset/1 -> DedicatedPID/2
  Error/1 -> DedicatedPID/1

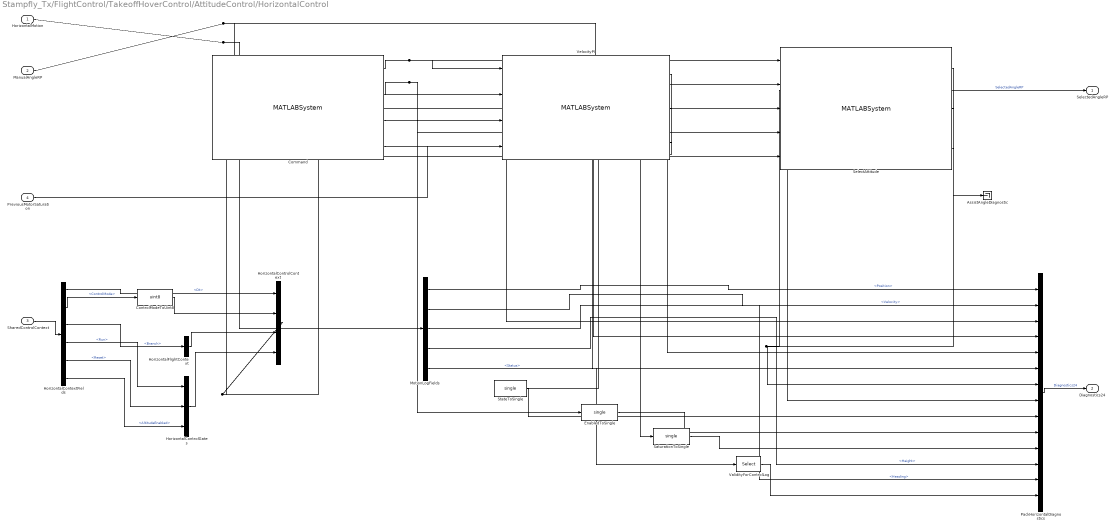
== system Stampfly_Tx/FlightControl/TakeoffHoverControl/AttitudeControl/HorizontalControl ==
  HorizontalMotion : Inport  Description=HorizontalMotion：水平推定・制御のデータと実行条件を選択・結合します。2軸の順序は局所X（基準機首）、Y（右）です。
  ManualAngleRP : Inport  Description=ManualAngleRP：水平推定・制御のデータと実行条件を選択・結合します。2軸の順序は局所X（基準機首）、Y（右）です。  Port=2
  SharedControlContext : Inport  Description=SharedControlContext：水平推定・制御のデータと実行条件を選択・結合します。2軸の順序は局所X（基準機首）、Y（右）です。  Port=3
  PreviousMotorSaturation : Inport  Description=PreviousMotorSaturation：水平推定・制御のデータと実行条件を選択・結合します。2軸の順序は局所X（基準機首）、Y（右）です。  Port=4
  AssistAngleDiagnostic : Terminator
      settings: Description=AssistAngleDiagnostic：水平推定・制御のデータと実行条件を選択・結合します。2軸の順序は局所X（基準機首）、Y（右）です。
  Command : MATLABSystem  Description=|  System=horizontal.Command  Enabled=true  SampleTime=.0025  MaxSpeedMps=.3  CommandAccelerationMps2=.6  PositionGainPerS=.8  EngageHeightM=.20  ReleaseHeightM=.15  HealthyTimeS=.5  RecoveryTimeS=1.0  NeutralEnter=.05  NeutralExit=.08  StopSpeedMps=.08  StopTimeS=.3  ManualAngleLimitRad=pi / 6  SimulateUsing=Code generation
      | %COMMAND 概要：移動・減速・停止位置保持を切り替えて水平速度目標を作ります。
      |     % 既存のスティック中立補正済み角度を、水平補助中だけ速度指令へ解釈します。
      |     % 将来の自動移動は、この出力と同じ局所速度[m/s]を制御器へ渡せます。
      mask Type: horizontal.Command
  ControlModeToUint8 : DataTypeConversion  Description=ControlModeToUint8：水平推定・制御のデータと実行条件を選択・結合します。2軸の順序は局所X（基準機首）、Y（右）です。  OutDataTypeStr=uint8  SaturateOnIntegerOverflow=off  RndMeth=Floor
  EnabledToSingle : DataTypeConversion  Description=EnabledToSingle：水平推定・制御のデータと実行条件を選択・結合します。2軸の順序は局所X（基準機首）、Y（右）です。  OutDataTypeStr=single  SaturateOnIntegerOverflow=off  RndMeth=Floor
  HorizontalContextFields : BusSelector  Description=HorizontalContextFields：水平推定・制御のデータと実行条件を選択・結合します。2軸の順序は局所X（基準機首）、Y（右）です。  OutputSignals=Dt,ControlMode,FlightContext.Branch,ControlContext.Run,ControlContext.Reset,ControlContext.AltitudeEnabled
  HorizontalControlContext : BusCreator  Description=HorizontalControlContext：水平推定・制御のデータと実行条件を選択・結合します。2軸の順序は局所X（基準機首）、Y（右）です。  Inputs=4  OutDataTypeStr=Bus: HorizontalControlContextBus  NonVirtualBus=on
      settings: InheritFromInputs=off
  HorizontalControlGates : BusCreator  Description=HorizontalControlGates：水平推定・制御のデータと実行条件を選択・結合します。2軸の順序は局所X（基準機首）、Y（右）です。  Inputs=3  OutDataTypeStr=Bus: HorizontalControlGatesBus  NonVirtualBus=on
      settings: InheritFromInputs=off
  HorizontalFlightContext : BusCreator  Description=HorizontalFlightContext：水平推定・制御のデータと実行条件を選択・結合します。2軸の順序は局所X（基準機首）、Y（右）です。  Inputs=1  OutDataTypeStr=Bus: HorizontalFlightContextBus  NonVirtualBus=on
      settings: InheritFromInputs=off
  MotionLogFields : BusSelector  Description=MotionLogFields：水平推定・制御のデータと実行条件を選択・結合します。2軸の順序は局所X（基準機首）、Y（右）です。  OutputSignals=Position,Velocity,Heading,Height,Status
  PackHorizontalDiagnostics : Mux  Description=PackHorizontalDiagnostics：水平推定・制御のデータと実行条件を選択・結合します。2軸の順序は局所X（基準機首）、Y（右）です。  Inputs=14
  SaturationToSingle : DataTypeConversion  Description=SaturationToSingle：水平推定・制御のデータと実行条件を選択・結合します。2軸の順序は局所X（基準機首）、Y（右）です。  OutDataTypeStr=single  SaturateOnIntegerOverflow=off  RndMeth=Floor
  SelectAttitude : MATLABSystem  Description=|  System=horizontal.SelectAttitude  SampleTime=.0025  EngageTimeS=.3  ReleaseTimeS=.15  MaxAssistTiltDeg=10  MaxAssistTiltRateDegps=20  SimulateUsing=Code generation
      | %SELECTATTITUDE 概要：水平補助と従来の姿勢目標を滑らかに切り替えます。
      |     % 補助OFFでBlend=0なら元のsingle値をそのまま返し、従来出力を保ちます。
      |             % 1. 有効な水平加速度を、既存の制御座標のRoll/Pitchへ戻します。
      mask Type: horizontal.SelectAttitude
  StateToSingle : DataTypeConversion  Description=StateToSingle：水平推定・制御のデータと実行条件を選択・結合します。2軸の順序は局所X（基準機首）、Y（右）です。  OutDataTypeStr=single  SaturateOnIntegerOverflow=off  RndMeth=Floor
  ValidityForControlLog : Selector  Description=ValidityForControlLog：水平推定・制御のデータと実行条件を選択・結合します。2軸の順序は局所X（基準機首）、Y（右）です。  InputPortWidth=8  IndexOptions=Index vector (dialog)  Indices=[1 4 5 7]  OutputSizes=1
  VelocityPI : MATLABSystem  Description=|  System=horizontal.VelocityPI  SampleTime=.0025  ProportionalGainPerS=1.8  IntegralGainPerS2=.5  MaxAccelerationMps2=.6  IntegralLimitMps2=.25  AccelerationSlewMps3=2.0  SimulateUsing=Code generation
      | %VELOCITYPI 概要：局所水平速度の誤差をPIで水平加速度へ変換します。
      |     % 50 Hzの有効な観測だけ積分し、欠測・解除時は積分をリセットします。
      |     % 速度指令の出所を持たないため、将来の自動移動にも同じ境界を使えます。
      mask Type: horizontal.VelocityPI
  SelectedAngleRP : Outport  Description=SelectedAngleRP：水平推定・制御のデータと実行条件を選択・結合します。2軸の順序は局所X（基準機首）、Y（右）です。
  Diagnostics24 : Outport  Description=Diagnostics24：水平推定・制御のデータと実行条件を選択・結合します。2軸の順序は局所X（基準機首）、Y（右）です。  Port=2
  wires:
  SharedControlContext/1 -> HorizontalContextFields/1
  MotionLogFields/5 -> ValidityForControlLog/1  "<Status>"
  ControlModeToUint8/1 -> HorizontalControlContext/2
  HorizontalContextFields/5 -> HorizontalControlGates/2  "<Reset>"
  Command/1 -> PackHorizontalDiagnostics/3, VelocityPI/1
  HorizontalContextFields/3 -> HorizontalFlightContext/1  "<Branch>"
  PackHorizontalDiagnostics/1 -> Diagnostics24/1  "Diagnostics24"
  HorizontalContextFields/1 -> HorizontalControlContext/1  "<Dt>"
  Command/2 -> EnabledToSingle/1, SelectAttitude/4, VelocityPI/3
  HorizontalContextFields/6 -> HorizontalControlGates/3  "<AltitudeEnabled>"
  HorizontalContextFields/4 -> HorizontalControlGates/1  "<Run>"
  HorizontalControlGates/1 -> HorizontalControlContext/4
  HorizontalContextFields/2 -> ControlModeToUint8/1  "<ControlMode>"
  Command/3 -> StateToSingle/1
  HorizontalFlightContext/1 -> HorizontalControlContext/3
  ManualAngleRP/1 -> SelectAttitude/1, Command/2
  HorizontalMotion/1 -> SelectAttitude/3, MotionLogFields/1, VelocityPI/2, Command/1
  HorizontalControlContext/1 -> SelectAttitude/5, Command/3
  MotionLogFields/2 -> PackHorizontalDiagnostics/2  "<Velocity>"
  Command/4 -> PackHorizontalDiagnostics/4
  MotionLogFields/1 -> PackHorizontalDiagnostics/1  "<Position>"
  EnabledToSingle/1 -> PackHorizontalDiagnostics/10
  PreviousMotorSaturation/1 -> VelocityPI/4
  VelocityPI/1 -> PackHorizontalDiagnostics/5, SelectAttitude/2
  VelocityPI/2 -> PackHorizontalDiagnostics/6
  VelocityPI/3 -> SaturationToSingle/1
  MotionLogFields/3 -> PackHorizontalDiagnostics/13  "<Heading>"
  MotionLogFields/4 -> PackHorizontalDiagnostics/12  "<Height>"
  StateToSingle/1 -> PackHorizontalDiagnostics/9
  SaturationToSingle/1 -> PackHorizontalDiagnostics/11
  SelectAttitude/1 -> SelectedAngleRP/1, PackHorizontalDiagnostics/7  "SelectedAngleRP"
  SelectAttitude/2 -> PackHorizontalDiagnostics/8
  SelectAttitude/3 -> AssistAngleDiagnostic/1
  ValidityForControlLog/1 -> PackHorizontalDiagnostics/14

== system Stampfly_Tx/FlightControl/TakeoffHoverControl/AttitudeControl/PitchAnglePID ==
  Error : Inport
  Dt : Inport  Port=2
  Reset : Inport  Port=3
  Enable : EnablePort
  DedicatedPID : slpidlib/PID Controller  Description=飛行比較用の専用PID。Ideal形式、台形積分・微分フィルター、実測Dt、単精度。  Controller=PID  Form=Ideal  TimeDomain=Discrete-time  UseExternalTs=on  SampleTime=.0025  IntegratorMethod=Trapezoidal  FilterMethod=Trapezoidal  ControllerParametersSource=internal  P=single(5)  I=single(1)/single(4)  UseKiTs=off  D=single(0.039999999105930328)  UseExternalDerivativeSource=off  N=single(1)/(single(0.125)*single(0.039999999105930328))  UseFilter=on  TunerSelectOption=Transfer Function Based (PID Tuner App)  InitialConditionSource=external  InitialConditionForIntegrator=0  InitialConditionForFilter=0  DifferentiatorICPrevScaledInput=0  ExternalReset=level  TrackingMode=off  Kt=1  LimitOutput=off  SatLimitsSource=internal  UpperSaturationLimit=inf  LowerSaturationLimit=-inf  LinearizeAsGain=off  AntiWindupMode=none  Kb=1  LimitIntegrator=on  UpperIntegratorSaturationLimit=single(30000)  LowerIntegratorSaturationLimit=single(-30000)  PGainOutDataTypeStr=single  PProdOutDataTypeStr=single  POutMin=[]  POutMax=[]  IGainOutDataTypeStr=single  IProdOutDataTypeStr=single  IOutMin=[]  IOutMax=[]  DGainOutDataTypeStr=single  DProdOutDataTypeStr=single  DOutMin=[]  DOutMax=[]  NGainOutDataTypeStr=single  NProdOutDataTypeStr=single  NOutMin=[]  NOutMax=[]  SumOutDataTypeStr=single  SumOutMin=[]  SumOutMax=[]  SaturationOutDataTypeStr=single  SaturationOutMin=[]  SaturationOutMax=[]  PParamDataTypeStr=single  PParamMin=[]  PParamMax=[]  IParamDataTypeStr=single  IParamMin=[]  IParamMax=[]  DParamDataTypeStr=single  DParamMin=[]  DParamMax=[]  NParamDataTypeStr=single  NParamMin=[]  NParamMax=[]  KbParamDataTypeStr=single  KbParamMin=[]  KbParamMax=[]  KtParamDataTypeStr=single  KtParamMin=[]  KtParamMax=[]  KbOutDataTypeStr=single  KbOutMin=[]  KbOutMax=[]  KtOutDataTypeStr=single  KtOutMin=[]  KtOutMax=[]  IntegratorOutDataTypeStr=single  IntegratorOutMin=[]  IntegratorOutMax=[]  FilterOutDataTypeStr=single  FilterOutMin=[]  FilterOutMax=[]  SumI1OutDataTypeStr=single  SumI1OutMin=[]  SumI1OutMax=[]  SumI2OutDataTypeStr=single  SumI2OutMin=[]  SumI2OutMax=[]  SumI3OutDataTypeStr=single  SumI3OutMin=[]  SumI3OutMax=[]  SumI4OutDataTypeStr=single  SumI4OutMin=[]  SumI4OutMax=[]  SumDOutDataTypeStr=single  SumDOutMin=[]  SumDOutMax=[]  SumAccumDataTypeStr=single  SumI1AccumDataTypeStr=single  SumI2AccumDataTypeStr=single  SumI3AccumDataTypeStr=single  SumI4AccumDataTypeStr=single  SumDAccumDataTypeStr=single  DifferentiatorOutDataTypeStr=single  DifferentiatorOutMin=[]  DifferentiatorOutMax=[]  FilterDiffOutCoefMin=[]  FilterDiffOutCoefMax=[]  ReciprocalOutDataTypeStr=single  ReciprocalOutMin=[]  ReciprocalOutMax=[]  SumDenOutDataTypeStr=single  SumDenOutMin=[]  SumDenOutMax=[]  SumNumOutDataTypeStr=single  SumNumOutMin=[]  SumNumOutMax=[]  SumDenAccumDataTypeStr=single  SumNumAccumDataTypeStr=single  DivideOutDataTypeStr=single  DivideOutMin=[]  DivideOutMax=[]  UdiffTsProdOutDataTypeStr=single  UdiffTsProdOutMin=[]  UdiffTsProdOutMax=[]  NTsProdOutDataTypeStr=single  NTsProdOutMin=[]  NTsProdOutMax=[]  UintegralTsProdOutDataTypeStr=single  UintegralTsProdOutMin=[]  UintegralTsProdOutMax=[]  UngainTsProdOutDataTypeStr=single  UngainTsProdOutMin=[]  UngainTsProdOutMax=[]  ClampingZeroOutDataTypeStr=single  ClampingZeroOutMin=[]  ClampingZeroOutMax=[]  FilterDenConstantOutDataTypeStr=single  FilterDenConstantOutMin=[]  FilterDenConstantOutMax=[]  PCopyOutDataTypeStr=single  PCopyOutMin=[]  PCopyOutMax=[]  NCopyOutDataTypeStr=single  NCopyOutMin=[]  NCopyOutMax=[]  IntegratorContinuousStateAttributes=''  IntegratorStateMustResolveToSignalObject=off  IntegratorRTWStateStorageClass=Auto  FilterContinuousStateAttributes=''  FilterStateMustResolveToSignalObject=off  FilterRTWStateStorageClass=Auto  ParallelPVariant=Passthrough  IdealPVariant=InternalParameters  IVariant=InternalParameters  DVariant=InternalParameters  IntegratorVariant=Discrete  SatVariant=Disabled  AWVariant=Passthrough  PCopyVariant=Disabled  TRVariant=Disabled  FdbkBlocksVariant=Forward  IdealPFdbkVariant=Disabled  SatFdbkVariant=Disabled  DerivativeFilterVariant=TrapezoidalFilter  NVariant=InternalParameters  NCopyVariant=InternalParameters  FilterICVariant=ExternalICs  IntegratorICVariant=ExternalICs  ExternalResetVariant=ExternalReset  TRSumVariant=Passthrough  SumFdbkVariant=Disabled  SumVariant=Sum_PID  TsampFilterVariant=ExternalTs  TsampNgainVariant=Passthrough  TsampIntegralVariant=ExternalTs  ExternalSaturationOutDataTypeStr=Inherit: Same as second input  DerivativeSourceVariant=ErrorSignal  PreIntVariant=InternalPreInt
      settings: LibrarySourceBlock=simulink/Discrete/Discrete PID Controller
  ZeroInitialCondition : Constant  Description=ZeroInitialCondition：固定値 single(0) を出力します。意味と単位は親の機能説明と信号名を参照します。  Value=single(0)
  Output : Outport
  wires:
  DedicatedPID/1 -> Output/1
  Dt/1 -> DedicatedPID/5
  ZeroInitialCondition/1 -> DedicatedPID/4, DedicatedPID/3
  Reset/1 -> DedicatedPID/2
  Error/1 -> DedicatedPID/1
